simulink model "Progetto_LQR_simulink"  (R2026a)
settings: Solver=ode23t  StopTime=4  MaxStep=0.0050000000000000001  RelTol=1.0000000000000001e-05  AbsTol=9.9999999999999995e-08
InitFcn:
  | actuator = actuator_params_nominal();
  | [Gact, info] = build_nominal_actuator(actuator);
  | 
  | % Parametri del robot
  | p = sea_params_nominal();
  | Simulink.Bus.createObject(p);
  | 
  | % Equilibrio desiderato
  | qbar = [pi/2; 0];
  | 
  | % Calcolo stato e coppia di equilibrio
  | [xbar, taubar, info] = sea_static_equilibrium(qbar, p);
undefined symbols (not defined in the file): A, B, C, K, L, Nr, taubar, xbar
libraries: cstblocks_lti x2
Description:
  | explicit LQR plus Kalman observer -> M3 actuators -> nonlinear M1 SEA
settings Model: Creator=aless  LastModifiedBy=rebec

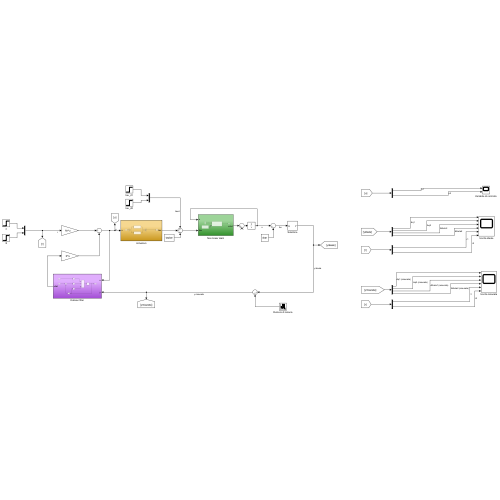
[thumbnail: Simulink's stored preview of the top-level diagram]
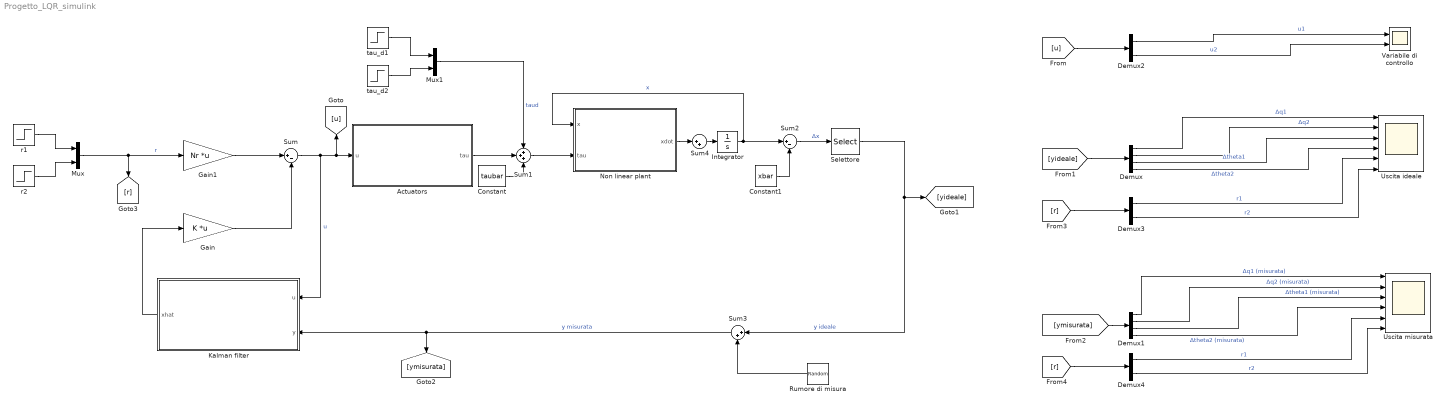
== system Progetto_LQR_simulink ==
  Actuators : Subsystem
  Constant : Constant  Value=taubar
  Constant1 : Constant  Value=xbar
  Demux : Demux
  Demux1 : Demux
  Demux2 : Demux  Outputs=2
  Demux3 : Demux  Outputs=2
  Demux4 : Demux  Outputs=2
  Gain : Gain  Gain=K  Multiplication=Matrix(K*u)
  Gain1 : Gain  Gain=Nr  Multiplication=Matrix(K*u)
  Integrator : Integrator  InitialCondition=xbar
  Kalman filter : Subsystem
  Mux : Mux  Inputs=2
  Mux1 : Mux  Inputs=2
  Non linear plant : Subsystem
  Rumore di misura : RandomNumber  Variance=(0.05*pi/180)^2  Seed=20260826  SampleTime=0.002
  Selettore : Selector  InputPortWidth=8  IndexOptions=Index vector (dialog)  Indices=[1 2 5 6]  OutputSizes=1
  Sum : Sum  Inputs=|+-
  Sum1 : Sum  Inputs=+++
  Sum2 : Sum  Inputs=|+-
  Sum3 : Sum  Inputs=|++
  Sum4 : Sum  Inputs=|++
  Uscita ideale : Scope  NumInputPorts=6
      settings: Title=y (uscita ideale)  ActiveDisplayYMinimum=-0.2641427698556385  ActiveDisplayYMaximum=0.37201372594716681
  Uscita misurata : Scope  NumInputPorts=6
      settings: Title=y (uscita ideale)  ActiveDisplayYMinimum=-0.11442029066688837  ActiveDisplayYMaximum=0.16914890182413583
  Variabile di controllo : Scope  NumInputPorts=2
      settings: ActiveDisplayYMinimum=-2.6959450601265313  ActiveDisplayYMaximum=5.9059369724787079  DataLoggingVariableName=ScopeData2
  r1 : Step  FinalValue=5*pi/180  SampleTime=0
  r2 : Step  FinalValue=0  SampleTime=0
  tau_d1 : Step  FinalValue=0.5  SampleTime=0
  tau_d2 : Step  FinalValue=0  SampleTime=0
  wires:
  Integrator/1 -> Non linear plant/1(x), Sum2/1  "x"
  Gain1/1 -> Sum/1
  Gain/1 -> Sum/2
  Sum/1 -> Kalman filter/1(u), [u], Actuators/1(u)  "u"
  r1/1 -> Mux/1
  r2/1 -> Mux/2
  Mux/1 -> [r], Gain1/1  "r"
  Sum1/1 -> Non linear plant/2(tau)
  Constant1/1 -> Sum2/2
  Sum2/1 -> Selettore/1  "Δx"
  Kalman filter/1(xhat) -> Gain/1
  Selettore/1 -> [yideale], Sum3/1  "y ideale"
  Non linear plant/1(xdot) -> Sum4/1
  Sum4/1 -> Integrator/1
  Demux/1 -> Uscita ideale/1  "Δq1"
  Demux/2 -> Uscita ideale/2  "Δq2"
  Demux/3 -> Uscita ideale/3  "Δtheta1"
  Demux/4 -> Uscita ideale/4  "Δtheta2"
  Demux1/2 -> Uscita misurata/2  "Δq2 (misurata)"
  Demux1/4 -> Uscita misurata/4  "Δtheta2 (misurata)"
  Demux1/1 -> Uscita misurata/1  "Δq1 (misurata)"
  Demux1/3 -> Uscita misurata/3  "Δtheta1 (misurata)"
  Sum3/1 -> Kalman filter/2(y), [ymisurata]  "y misurata"
  Demux2/1 -> Variabile di controllo/1  "u1"
  Demux2/2 -> Variabile di controllo/2  "u2"
  Rumore di misura/1 -> Sum3/2
  [u] -> Demux2/1
  [yideale] -> Demux/1
  [ymisurata] -> Demux1/1
  [r] -> Demux3/1
  [r] -> Demux4/1
  Demux3/1 -> Uscita ideale/5  "r1"
  Demux3/2 -> Uscita ideale/6  "r2"
  Demux4/1 -> Uscita misurata/5  "r1"
  Demux4/2 -> Uscita misurata/6  "r2"
  tau_d2/1 -> Mux1/2
  tau_d1/1 -> Mux1/1
  Mux1/1 -> Sum1/1  "taud"
  Constant/1 -> Sum1/3
  Actuators/1(tau) -> Sum1/2

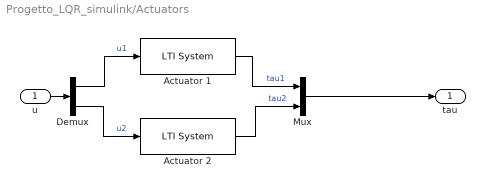
== system Progetto_LQR_simulink/Actuators ==
  u : Inport
  Actuator 1 : cstblocks_lti/LTI System  sys=Gact  IC=[]  PadeOrder=0
      settings: LibrarySourceBlock=cstblocks/LTI System
  Actuator 2 : cstblocks_lti/LTI System  sys=Gact  IC=[]  PadeOrder=0
      settings: LibrarySourceBlock=cstblocks/LTI System
  Demux : Demux  Outputs=2
  Mux : Mux  Inputs=2
  tau : Outport
  wires:
  Actuator 2/1 -> Mux/2  "tau2"
  Demux/2 -> Actuator 2/1  "u2"
  u/1 -> Demux/1
  Demux/1 -> Actuator 1/1  "u1"
  Mux/1 -> tau/1
  Actuator 1/1 -> Mux/1  "tau1"

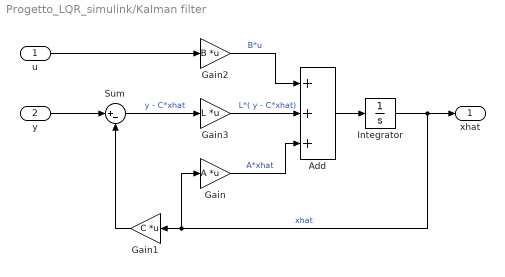
== system Progetto_LQR_simulink/Kalman filter ==
  u : Inport
  y : Inport  Port=2
  Add : Sum  Inputs=+++
  Gain : Gain  Gain=A  Multiplication=Matrix(K*u)
  Gain1 : Gain  Gain=C  Multiplication=Matrix(K*u)
  Gain2 : Gain  Gain=B  Multiplication=Matrix(K*u)
  Gain3 : Gain  Gain=L  Multiplication=Matrix(K*u)
  Integrator : Integrator
  Sum : Sum  Inputs=|+-
  xhat : Outport
  wires:
  u/1 -> Gain2/1
  y/1 -> Sum/1
  Gain1/1 -> Sum/2
  Sum/1 -> Gain3/1  "y - C*xhat"
  Gain3/1 -> Add/2  "L*( y - C*xhat)"
  Gain2/1 -> Add/1  "B*u"
  Gain/1 -> Add/3  "A*xhat"
  Add/1 -> Integrator/1
  Integrator/1 -> Gain/1, Gain1/1, xhat/1  "xhat"

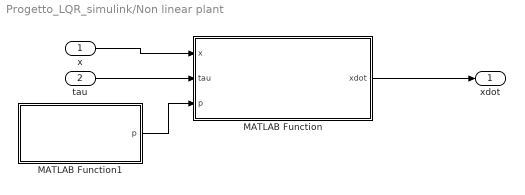
== system Progetto_LQR_simulink/Non linear plant ==
  x : Inport
  tau : Inport  Port=2
  MATLAB Function : MATLAB Function  TreatAsAtomicUnit=on
  MATLAB Function1 : MATLAB Function  TreatAsAtomicUnit=on
  xdot : Outport
  wires:
  x/1 -> MATLAB Function/1(x)
  tau/1 -> MATLAB Function/2(tau)
  MATLAB Function/1(xdot) -> xdot/1
  MATLAB Function1/1(p) -> MATLAB Function/3(p)

== matlab function Progetto_LQR_simulink/Non linear plant/MATLAB Function ==
  data: x input; xdot output; tau input; p input
function xdot = sea_nonlinear_rhs(x, tau, p)
%SEA_NONLINEAR_RHS Full eight-state nonlinear dynamics of the 2R SEA robot.
%   X = [q; qdot; theta; thetadot] is an 8-by-1 state vector and TAU is
%   the 2-by-1 motor torque in N*m. The output follows the same state order.

assert(numel(x) == 8, 'sea_nonlinear_rhs:InvalidState', ...
    'The state must contain exactly eight elements.');
assert(numel(tau) == 2, 'sea_nonlinear_rhs:InvalidInput', ...
    'The motor torque must contain exactly two elements.');

x = reshape(x, 8, 1);
tau = reshape(tau, 2, 1);

q = x(1:2);
qdot = x(3:4);
theta = x(5:6);
thetadot = x(7:8);

M = sea_link_inertia(q, p);
C = sea_coriolis(q, qdot, p);
G = sea_gravity(q, p);
tauElastic = sea_elastic_torque(q, theta, p);

qddot = M \ (tauElastic - C * qdot - G);
thetaddot = p.Jm \ (tau - p.Bm * thetadot - tauElastic);

xdot = [qdot; qddot; thetadot; thetaddot];
end

== matlab function Progetto_LQR_simulink/Non linear plant/MATLAB Function1 ==
  data: p output Bus: slBus1
function p = sea_params_nominal
%SEA_PARAMS_NOMINAL Nominal mechanical parameters of the 2R SEA robot.
%   P = SEA_PARAMS_NOMINAL returns the values stated by the official
%   assignment. Matrices follow the joint order [joint 1; joint 2].

p.m1 = 1.0;                   % kg
p.m2 = 0.8;                   % kg
p.l1 = 0.4;                   % m
p.l2 = 0.3;                   % m
p.Jm = diag([0.01, 0.01]);    % kg*m^2
p.Bm = diag([0.02, 0.02]);    % N*m*s/rad
p.Ks = diag([50, 40]);        % N*m/rad
p.g = 9.81;                   % m/s^2
end
